simulink model "Aman_plant"  (R2025a)
settings: Solver=VariableStepAuto  StartTime=0.0  StopTime=10.0  RelTol=1e-3
undefined symbols (not defined in the file): magnitude
libraries: simulink_extras x1
settings Model: Creator=amansharma  LastModifiedBy=amansharma

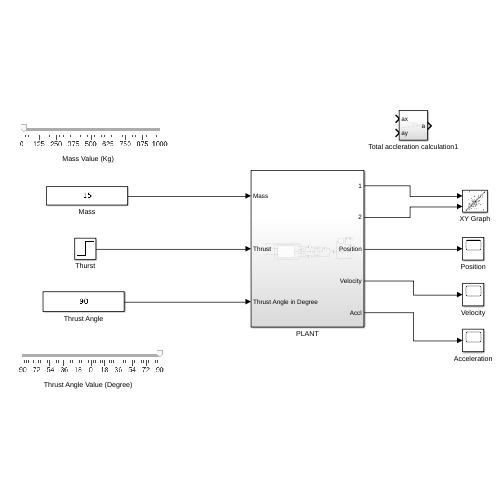
[thumbnail: Simulink's stored preview of the top-level diagram]
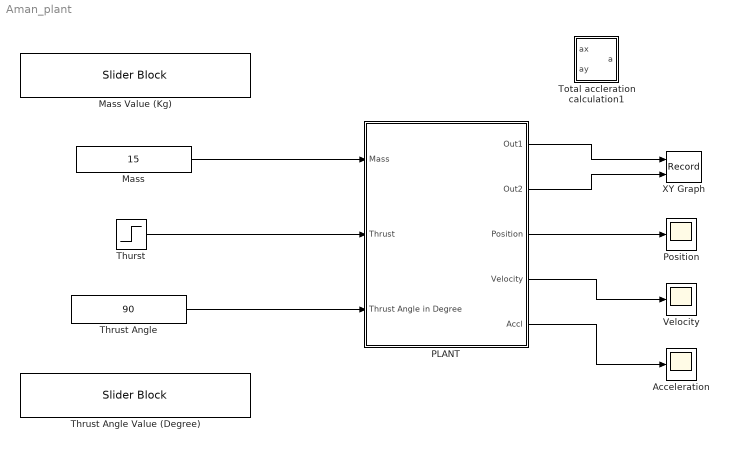
== system Aman_plant ==
  Acceleration : Scope
      settings: ActiveDisplayYMinimum=-1  ActiveDisplayYMaximum=1
  Mass : Constant  Value=15
  Mass Value (Kg) : SliderBlock  LabelPosition=Hide  ScaleMax=1000
  PLANT : Subsystem
  Position : Scope
      settings: ActiveDisplayYMinimum=-1  ActiveDisplayYMaximum=1  DataLoggingVariableName=ScopeData2
  Thrust Angle : Constant  Value=90
  Thrust Angle Value (Degree) : SliderBlock  LabelPosition=Hide  ScaleMin=-90  ScaleMax=90
  Thurst : Step  SampleTime=0
  Total accleration calculation1 : Subsystem
  Velocity : Scope
      settings: ActiveDisplayYMinimum=-110.34194116193835  ActiveDisplayYMaximum=12.260215684659814
  XY Graph : Record  NumPorts=2.0  FileSettingsInternal="{\"entries\":[{\"content\":{\"excelSettings\":{\"content\":{},\"type\":\"Streamout.ExcelSettings\"},\"parquetSettings\":{\"content\":{},\"type\":\"Streamout.ParquetSettings\"}},\"type\":\"Streamout.FileSettingStorage\",\"uuid\":\"\"}],\"packageUris\":[\"http:\\/\\/schema.mathworks.com\\/mf0\\/streamout_blocks\\/R2020a\"],\"version\":\"1.0\"}"  FrameSettings=[0, 0]  Layout=[1 1]  SignalsInternal="{\"entries\":[{\"content\":{},\"type\":\"RecordBlkView.InputSignals\",\"uuid\":\"\"}],\"packageUris\":[\"http:\\/\\/schema.mathworks.com\\/mf0\\/streamout_blocks\\/R2020a\"],\"version\":\"1.0\"}"  VisualizationBindings="{\"sparklinesplugin\":{\"info\":[{\"bindingParametersList\":[],\"subplotID\":1}]}}"  CompatibilityTag=XY
  wires:
  Mass/1 -> PLANT/1(Mass)
  Thurst/1 -> PLANT/2(Thrust)
  Thrust Angle/1 -> PLANT/3(Thrust Angle in Degree)
  PLANT/1(Out1) -> XY Graph/1
  PLANT/2(Out2) -> XY Graph/2
  PLANT/3(Position) -> Position/1
  PLANT/4(Velocity) -> Velocity/1
  PLANT/5(Accl) -> Acceleration/1

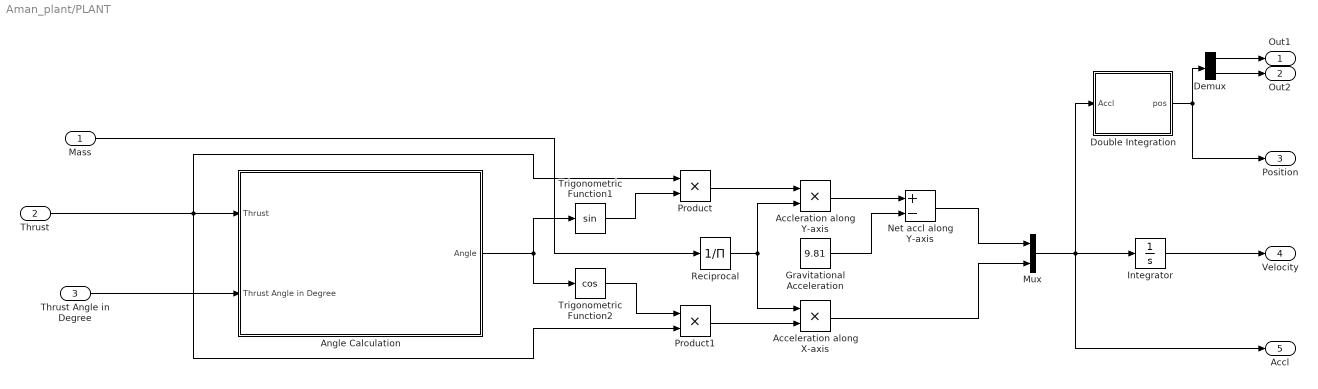
== system Aman_plant/PLANT ==
  Mass : Inport
  Thrust : Inport  Port=2
  Thrust Angle in Degree : Inport  Port=3
  " Gravitational Acceleration" : Constant  Value=9.81
  Acceleration along X-axis : Product
  Accleration along Y-axis : Product
  Angle Calculation : Subsystem
  Demux : Demux  Outputs=2
  Double Integration : Subsystem
  Integrator : Integrator
  Mux : Mux  Inputs=2
  Net accl along Y-axis : Sum  Inputs=+-
  Product : Product
  Product1 : Product
  Reciprocal : Product  Inputs=/
  Trigonometric Function1 : Trigonometry
  Trigonometric Function2 : Trigonometry  Operator=cos
  Out1 : Outport
  Out2 : Outport  Port=2
  Position : Outport  Port=3
  Velocity : Outport  Port=4
  Accl : Outport  Port=5
  wires:
  Mass/1 -> Reciprocal/1
  Thrust Angle in Degree/1 -> Angle Calculation/2(Thrust Angle in Degree)
  Angle Calculation/1(Angle) -> Trigonometric Function2/1, Trigonometric Function1/1
  Acceleration along X-axis/1 -> Mux/2
  Accleration along Y-axis/1 -> Net accl along Y-axis/1
  Integrator/1 -> Velocity/1
  Product/1 -> Accleration along Y-axis/1
  " Gravitational Acceleration"/1 -> Net accl along Y-axis/2
  Net accl along Y-axis/1 -> Mux/1
  Reciprocal/1 -> Acceleration along X-axis/1, Accleration along Y-axis/2
  Double Integration/1(pos) -> Position/1, Demux/1
  Demux/2 -> Out2/1
  Mux/1 -> Accl/1, Double Integration/1(Accl), Integrator/1
  Demux/1 -> Out1/1
  Thrust/1 -> Product1/2, Product/1, Angle Calculation/1(Thrust)
  Trigonometric Function1/1 -> Product/2
  Product1/1 -> Acceleration along X-axis/2
  Trigonometric Function2/1 -> Product1/1

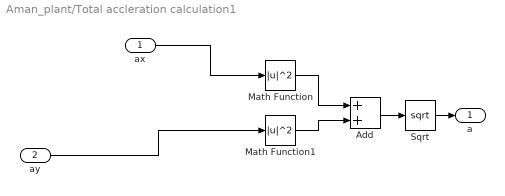
== system Aman_plant/Total accleration calculation1 ==
  ax : Inport
  ay : Inport  Port=2
  Add : Sum
  Math Function : Math  Operator=magnitude^2
  Math Function1 : Math  Operator=magnitude^2
  Sqrt : Sqrt
  a : Outport
  wires:
  Math Function/1 -> Add/1
  Math Function1/1 -> Add/2
  Add/1 -> Sqrt/1
  ay/1 -> Math Function1/1
  Sqrt/1 -> a/1
  ax/1 -> Math Function/1

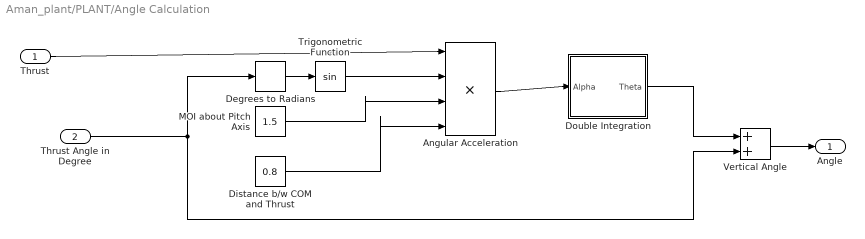
== system Aman_plant/PLANT/Angle Calculation ==
  Thrust : Inport
  Thrust Angle in Degree : Inport  Port=2
  "Angular Acceleration " : Product  Inputs=4
  Degrees to Radians : simulink_extras/Transformations/Degrees to Radians
  Distance b/w COM and Thrust : Constant  Value=0.8
  Double Integration : Subsystem
  MOI about Pitch Axis : Constant  Value=1.5
  Trigonometric Function : Trigonometry
  Vertical Angle : Sum
  Angle : Outport
  wires:
  "Angular Acceleration "/1 -> Double Integration/1(Alpha)
  MOI about Pitch Axis/1 -> "Angular Acceleration "/3
  Degrees to Radians/1 -> Trigonometric Function/1
  Vertical Angle/1 -> Angle/1
  Thrust Angle in Degree/1 -> Degrees to Radians/1, Vertical Angle/2
  Double Integration/1(Theta) -> Vertical Angle/1
  Trigonometric Function/1 -> "Angular Acceleration "/2
  Distance b/w COM and Thrust/1 -> "Angular Acceleration "/4
  Thrust/1 -> "Angular Acceleration "/1

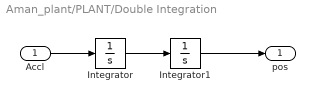
== system Aman_plant/PLANT/Double Integration ==
  Accl : Inport
  Integrator : Integrator
  Integrator1 : Integrator
  pos : Outport
  wires:
  Integrator/1 -> Integrator1/1
  Accl/1 -> Integrator/1
  Integrator1/1 -> pos/1

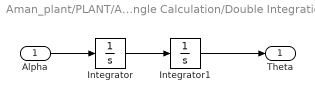
== system Aman_plant/PLANT/Angle Calculation/Double Integration ==
  Alpha : Inport
  Integrator : Integrator
  Integrator1 : Integrator
  Theta : Outport
  wires:
  Integrator/1 -> Integrator1/1
  Alpha/1 -> Integrator/1
  Integrator1/1 -> Theta/1
